simulink model "schuler1"  (Simulink 5.0)
settings: Solver=ode45  StartTime=0.0  StopTime=84*60  RelTol=1e-3
libraries: simulink x3
settings Model: Creator=mcar  LastModifiedBy=mcarroll  ExtModeAutoUpdateStatusClock=off  BlockReductionOpt=off  BooleanDataType=off

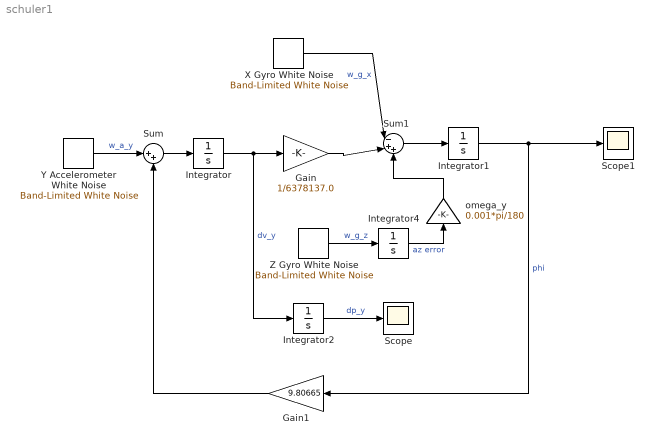
== system schuler1 ==
  Gain : Gain  Gain=1/6378137.0  SaturateOnIntegerOverflow=on
  Gain1 : Gain  Orientation=left  Gain=9.80665  SaturateOnIntegerOverflow=on
  Integrator{,1..2,4} (4 alike) : Integrator
  Scope : Scope
      settings: YMax=2  SampleInput=on  SampleTime=10
  Scope1 : Scope
      settings: TimeRange=12000  YMin=-0.02  YMax=0.12
  Sum : Sum  Inputs=|++  SaturateOnIntegerOverflow=on  InputSameDT=on
  Sum1 : Sum  Inputs=|-++  SaturateOnIntegerOverflow=on  InputSameDT=on
  X Gyro White Noise : simulink/Sources/Band-Limited White Noise  Cov=[(0.035*pi/180)^2]  Ts=0.1  seed=[23341]
  Y Accelerometer White Noise : simulink/Sources/Band-Limited White Noise  Cov=[0.1e-6/9.80665]  Ts=0.1  seed=[23341]
  Z Gyro White Noise : simulink/Sources/Band-Limited White Noise  Cov=[(0.035*pi/180^2)]  Ts=0.1  seed=[23341]
  omega_y : Gain  Orientation=up  Gain=0.001*pi/180  SaturateOnIntegerOverflow=on
  wires:
  Y Accelerometer White Noise/1 -> Sum/1  "w_a_y"
  Sum/1 -> Integrator/1
  Gain1/1 -> Sum/2
  Integrator/1 -> Gain/1, Integrator2/1  "dv_y"
  Integrator4/1 -> omega_y/1  "az error"
  Sum1/1 -> Integrator1/1
  Integrator2/1 -> Scope/1  "dp_y"
  Integrator1/1 -> Scope1/1, Gain1/1  "phi"
  Z Gyro White Noise/1 -> Integrator4/1  "w_g_z"
  X Gyro White Noise/1 -> Sum1/1  "w_g_x"
  omega_y/1 -> Sum1/3
  Gain/1 -> Sum1/2
